simulink model "s_c_nbe_m32k"  (R2018a)
settings: Solver=VariableStepDiscrete  StartTime=0.0  StopTime=1000  RelTol=1e-3
undefined symbols (not defined in the file): fft_stages, n_taps, output_bits, pfb_coeff_gen_calc, xengbits
libraries: xbsIndex_r4 x23714, casper_library_misc x17, xps_library x4, casper_library_scopes x4, xbsReplacements_r4 x4
(part 114 of 171)

== system s_c_nbe_m32k/DDC/dec_fir_async3/fir_col_async3/fir_tap8 ==
  a : Inport
  b : Inport  Port=2
  c : Inport  Port=3
  d : Inport  Port=4
  dv_in : Inport  Port=5
  AddSub0 : xbsIndex_r4/AddSub  mode=Addition  use_carryin=off  use_carryout=off  en=on  latency=add_latency  precision=Full  arith_type="Signed  (2's comp)"  n_bits=18  bin_pt=16  quantization=Truncate  overflow=Wrap  use_behavioral_HDL=on  hw_selection=Fabric  pipelined=off  use_rpm=on  dbl_ovrd=off  block_type=addsub
  AddSub1 : xbsIndex_r4/AddSub  mode=Addition  use_carryin=off  use_carryout=off  en=on  latency=add_latency  precision=Full  arith_type="Signed  (2's comp)"  n_bits=18  bin_pt=16  quantization=Truncate  overflow=Wrap  use_behavioral_HDL=on  hw_selection=Fabric  pipelined=off  use_rpm=on  dbl_ovrd=off  block_type=addsub
  Mult0 : xbsIndex_r4/Mult  precision=Full  arith_type="Signed  (2's comp)"  n_bits=18  bin_pt=17  quantization=Truncate  overflow=Wrap  en=on  latency=mult_latency  use_behavioral_HDL=on  opt=Speed  use_embedded=on  optimum_pipeline=off  pipeline=on  dbl_ovrd=off  use_rpm=off  placement_style=Rectangular shape  block_type=mult
  Mult1 : xbsIndex_r4/Mult  precision=Full  arith_type="Signed  (2's comp)"  n_bits=18  bin_pt=17  quantization=Truncate  overflow=Wrap  en=on  latency=mult_latency  use_behavioral_HDL=on  opt=Speed  use_embedded=on  optimum_pipeline=off  pipeline=on  dbl_ovrd=off  use_rpm=off  placement_style=Rectangular shape  block_type=mult
  Register{0..3} (4 alike) : xbsIndex_r4/Register  init=0  rst=off  en=on  dbl_ovrd=off  block_type=register
  coefficient : xbsIndex_r4/Constant  const=factor  gui_display_data_type=Fixed-point  arith_type=Signed (2's comp)  n_bits=coeff_bit_width  bin_pt=coeff_bin_pt  preci_type=Single  exp_width=8  frac_width=24  explicit_period=on  period=1  equ=P=C  opselect=C  inp2=PCIN>>17  opr=+  inp1=P  carry=CIN  dbl_ovrd=off  block_type=constant
  a_out : Outport
  b_out : Outport  Port=2
  c_out : Outport  Port=3
  d_out : Outport  Port=4
  real : Outport  Port=5
  imag : Outport  Port=6
  wires:
  dv_in/1 -> Register0/2, Register1/2, Register2/2, Register3/2, AddSub0/3, AddSub1/3, Mult0/3, Mult1/3
  d/1 -> AddSub1/2, Register3/1
  c/1 -> AddSub0/2, Register2/1
  b/1 -> AddSub1/1, Register1/1
  a/1 -> AddSub0/1, Register0/1
  Register0/1 -> a_out/1
  Register1/1 -> b_out/1
  Register2/1 -> c_out/1
  coefficient/1 -> Mult0/1, Mult1/1
  Register3/1 -> d_out/1
  AddSub0/1 -> Mult0/2
  Mult0/1 -> real/1
  AddSub1/1 -> Mult1/2
  Mult1/1 -> imag/1

== system s_c_nbe_m32k/DDC/dec_fir_async3/fir_col_async3/fir_tap9 ==
  a : Inport
  b : Inport  Port=2
  c : Inport  Port=3
  d : Inport  Port=4
  dv_in : Inport  Port=5
  AddSub0 : xbsIndex_r4/AddSub  mode=Addition  use_carryin=off  use_carryout=off  en=on  latency=add_latency  precision=Full  arith_type="Signed  (2's comp)"  n_bits=18  bin_pt=16  quantization=Truncate  overflow=Wrap  use_behavioral_HDL=on  hw_selection=Fabric  pipelined=off  use_rpm=on  dbl_ovrd=off  block_type=addsub
  AddSub1 : xbsIndex_r4/AddSub  mode=Addition  use_carryin=off  use_carryout=off  en=on  latency=add_latency  precision=Full  arith_type="Signed  (2's comp)"  n_bits=18  bin_pt=16  quantization=Truncate  overflow=Wrap  use_behavioral_HDL=on  hw_selection=Fabric  pipelined=off  use_rpm=on  dbl_ovrd=off  block_type=addsub
  Mult0 : xbsIndex_r4/Mult  precision=Full  arith_type="Signed  (2's comp)"  n_bits=18  bin_pt=17  quantization=Truncate  overflow=Wrap  en=on  latency=mult_latency  use_behavioral_HDL=on  opt=Speed  use_embedded=on  optimum_pipeline=off  pipeline=on  dbl_ovrd=off  use_rpm=off  placement_style=Rectangular shape  block_type=mult
  Mult1 : xbsIndex_r4/Mult  precision=Full  arith_type="Signed  (2's comp)"  n_bits=18  bin_pt=17  quantization=Truncate  overflow=Wrap  en=on  latency=mult_latency  use_behavioral_HDL=on  opt=Speed  use_embedded=on  optimum_pipeline=off  pipeline=on  dbl_ovrd=off  use_rpm=off  placement_style=Rectangular shape  block_type=mult
  Register{0..3} (4 alike) : xbsIndex_r4/Register  init=0  rst=off  en=on  dbl_ovrd=off  block_type=register
  coefficient : xbsIndex_r4/Constant  const=factor  gui_display_data_type=Fixed-point  arith_type=Signed (2's comp)  n_bits=coeff_bit_width  bin_pt=coeff_bin_pt  preci_type=Single  exp_width=8  frac_width=24  explicit_period=on  period=1  equ=P=C  opselect=C  inp2=PCIN>>17  opr=+  inp1=P  carry=CIN  dbl_ovrd=off  block_type=constant
  a_out : Outport
  b_out : Outport  Port=2
  c_out : Outport  Port=3
  d_out : Outport  Port=4
  real : Outport  Port=5
  imag : Outport  Port=6
  wires:
  dv_in/1 -> Register0/2, Register1/2, Register2/2, Register3/2, AddSub0/3, AddSub1/3, Mult0/3, Mult1/3
  d/1 -> AddSub1/2, Register3/1
  c/1 -> AddSub0/2, Register2/1
  b/1 -> AddSub1/1, Register1/1
  a/1 -> AddSub0/1, Register0/1
  Register0/1 -> a_out/1
  Register1/1 -> b_out/1
  Register2/1 -> c_out/1
  coefficient/1 -> Mult0/1, Mult1/1
  Register3/1 -> d_out/1
  AddSub0/1 -> Mult0/2
  Mult0/1 -> real/1
  AddSub1/1 -> Mult1/2
  Mult1/1 -> imag/1

== system s_c_nbe_m32k/DDC/dec_fir_async3/fir_col_async4/adder_tree1 ==
  sync : Inport
  din1 : Inport  Port=2
  din2 : Inport  Port=3
  din3 : Inport  Port=4
  din4 : Inport  Port=5
  din5 : Inport  Port=6
  din6 : Inport  Port=7
  din7 : Inport  Port=8
  din8 : Inport  Port=9
  din9 : Inport  Port=10
  din10 : Inport  Port=11
  din11 : Inport  Port=12
  din12 : Inport  Port=13
  din13 : Inport  Port=14
  din14 : Inport  Port=15
  din15 : Inport  Port=16
  din16 : Inport  Port=17
  addr{1..8} (8 alike) : xbsIndex_r4/AddSub  mode=Addition  use_carryin=off  use_carryout=off  en=off  latency=7  precision=Full  arith_type=Unsigned  n_bits=16  bin_pt=14  quantization=Truncate  overflow=Wrap  use_behavioral_HDL=on  hw_selection=DSP48  pipelined=on  use_rpm=on  dbl_ovrd=off  block_type=addsub
  addr{9..15} (7 alike) : xbsIndex_r4/AddSub  mode=Addition  use_carryin=off  use_carryout=off  en=off  latency=7  precision=Full  arith_type=Unsigned  n_bits=16  bin_pt=14  quantization=Truncate  overflow=Wrap  use_behavioral_HDL=off  hw_selection=DSP48  pipelined=on  use_rpm=on  dbl_ovrd=off  block_type=addsub
  sync_delay : xbsIndex_r4/Delay  rst=off  infoeditControl=Selection of Reset will increase slice count due to use of real FFs and instead of SRLs  en=off  latency=28  reg_retiming=on  dbl_ovrd=off  block_type=delay
      settings: block_version=11.4
  sync_out : Outport
  dout : Outport  Port=2
  wires:
  sync/1 -> sync_delay/1
  sync_delay/1 -> sync_out/1
  din1/1 -> addr1/1
  din2/1 -> addr1/2
  din3/1 -> addr2/1
  din4/1 -> addr2/2
  din5/1 -> addr3/1
  din6/1 -> addr3/2
  din7/1 -> addr4/1
  din8/1 -> addr4/2
  din9/1 -> addr5/1
  din10/1 -> addr5/2
  din11/1 -> addr6/1
  din12/1 -> addr6/2
  din13/1 -> addr7/1
  din14/1 -> addr7/2
  din15/1 -> addr8/1
  din16/1 -> addr8/2
  addr1/1 -> addr9/1
  addr2/1 -> addr9/2
  addr3/1 -> addr10/1
  addr4/1 -> addr10/2
  addr5/1 -> addr11/1
  addr6/1 -> addr11/2
  addr7/1 -> addr12/1
  addr8/1 -> addr12/2
  addr9/1 -> addr13/1
  addr10/1 -> addr13/2
  addr11/1 -> addr14/1
  addr12/1 -> addr14/2
  addr13/1 -> addr15/1
  addr14/1 -> addr15/2
  addr15/1 -> dout/1

== system s_c_nbe_m32k/DDC/dec_fir_async3/fir_col_async4/adder_tree2 ==
  sync : Inport
  din1 : Inport  Port=2
  din2 : Inport  Port=3
  din3 : Inport  Port=4
  din4 : Inport  Port=5
  din5 : Inport  Port=6
  din6 : Inport  Port=7
  din7 : Inport  Port=8
  din8 : Inport  Port=9
  din9 : Inport  Port=10
  din10 : Inport  Port=11
  din11 : Inport  Port=12
  din12 : Inport  Port=13
  din13 : Inport  Port=14
  din14 : Inport  Port=15
  din15 : Inport  Port=16
  din16 : Inport  Port=17
  addr{1..8} (8 alike) : xbsIndex_r4/AddSub  mode=Addition  use_carryin=off  use_carryout=off  en=off  latency=7  precision=Full  arith_type=Unsigned  n_bits=16  bin_pt=14  quantization=Truncate  overflow=Wrap  use_behavioral_HDL=on  hw_selection=DSP48  pipelined=on  use_rpm=on  dbl_ovrd=off  block_type=addsub
  addr{9..15} (7 alike) : xbsIndex_r4/AddSub  mode=Addition  use_carryin=off  use_carryout=off  en=off  latency=7  precision=Full  arith_type=Unsigned  n_bits=16  bin_pt=14  quantization=Truncate  overflow=Wrap  use_behavioral_HDL=off  hw_selection=DSP48  pipelined=on  use_rpm=on  dbl_ovrd=off  block_type=addsub
  sync_delay : xbsIndex_r4/Delay  rst=off  infoeditControl=Selection of Reset will increase slice count due to use of real FFs and instead of SRLs  en=off  latency=28  reg_retiming=on  dbl_ovrd=off  block_type=delay
      settings: block_version=11.4
  sync_out : Outport
  dout : Outport  Port=2
  wires:
  sync/1 -> sync_delay/1
  sync_delay/1 -> sync_out/1
  din1/1 -> addr1/1
  din2/1 -> addr1/2
  din3/1 -> addr2/1
  din4/1 -> addr2/2
  din5/1 -> addr3/1
  din6/1 -> addr3/2
  din7/1 -> addr4/1
  din8/1 -> addr4/2
  din9/1 -> addr5/1
  din10/1 -> addr5/2
  din11/1 -> addr6/1
  din12/1 -> addr6/2
  din13/1 -> addr7/1
  din14/1 -> addr7/2
  din15/1 -> addr8/1
  din16/1 -> addr8/2
  addr1/1 -> addr9/1
  addr2/1 -> addr9/2
  addr3/1 -> addr10/1
  addr4/1 -> addr10/2
  addr5/1 -> addr11/1
  addr6/1 -> addr11/2
  addr7/1 -> addr12/1
  addr8/1 -> addr12/2
  addr9/1 -> addr13/1
  addr10/1 -> addr13/2
  addr11/1 -> addr14/1
  addr12/1 -> addr14/2
  addr13/1 -> addr15/1
  addr14/1 -> addr15/2
  addr15/1 -> dout/1

== system s_c_nbe_m32k/DDC/dec_fir_async3/fir_col_async4/fir_tap1 ==
  a : Inport
  b : Inport  Port=2
  c : Inport  Port=3
  d : Inport  Port=4
  dv_in : Inport  Port=5
  AddSub0 : xbsIndex_r4/AddSub  mode=Addition  use_carryin=off  use_carryout=off  en=on  latency=add_latency  precision=Full  arith_type="Signed  (2's comp)"  n_bits=18  bin_pt=16  quantization=Truncate  overflow=Wrap  use_behavioral_HDL=on  hw_selection=Fabric  pipelined=off  use_rpm=on  dbl_ovrd=off  block_type=addsub
  AddSub1 : xbsIndex_r4/AddSub  mode=Addition  use_carryin=off  use_carryout=off  en=on  latency=add_latency  precision=Full  arith_type="Signed  (2's comp)"  n_bits=18  bin_pt=16  quantization=Truncate  overflow=Wrap  use_behavioral_HDL=on  hw_selection=Fabric  pipelined=off  use_rpm=on  dbl_ovrd=off  block_type=addsub
  Mult0 : xbsIndex_r4/Mult  precision=Full  arith_type="Signed  (2's comp)"  n_bits=18  bin_pt=17  quantization=Truncate  overflow=Wrap  en=on  latency=mult_latency  use_behavioral_HDL=on  opt=Speed  use_embedded=on  optimum_pipeline=off  pipeline=on  dbl_ovrd=off  use_rpm=off  placement_style=Rectangular shape  block_type=mult
  Mult1 : xbsIndex_r4/Mult  precision=Full  arith_type="Signed  (2's comp)"  n_bits=18  bin_pt=17  quantization=Truncate  overflow=Wrap  en=on  latency=mult_latency  use_behavioral_HDL=on  opt=Speed  use_embedded=on  optimum_pipeline=off  pipeline=on  dbl_ovrd=off  use_rpm=off  placement_style=Rectangular shape  block_type=mult
  Register{0..3} (4 alike) : xbsIndex_r4/Register  init=0  rst=off  en=on  dbl_ovrd=off  block_type=register
  coefficient : xbsIndex_r4/Constant  const=factor  gui_display_data_type=Fixed-point  arith_type=Signed (2's comp)  n_bits=coeff_bit_width  bin_pt=coeff_bin_pt  preci_type=Single  exp_width=8  frac_width=24  explicit_period=on  period=1  equ=P=C  opselect=C  inp2=PCIN>>17  opr=+  inp1=P  carry=CIN  dbl_ovrd=off  block_type=constant
  a_out : Outport
  b_out : Outport  Port=2
  c_out : Outport  Port=3
  d_out : Outport  Port=4
  real : Outport  Port=5
  imag : Outport  Port=6
  wires:
  dv_in/1 -> Register0/2, Register1/2, Register2/2, Register3/2, AddSub0/3, AddSub1/3, Mult0/3, Mult1/3
  d/1 -> AddSub1/2, Register3/1
  c/1 -> AddSub0/2, Register2/1
  b/1 -> AddSub1/1, Register1/1
  a/1 -> AddSub0/1, Register0/1
  Register0/1 -> a_out/1
  Register1/1 -> b_out/1
  Register2/1 -> c_out/1
  coefficient/1 -> Mult0/1, Mult1/1
  Register3/1 -> d_out/1
  AddSub0/1 -> Mult0/2
  Mult0/1 -> real/1
  AddSub1/1 -> Mult1/2
  Mult1/1 -> imag/1

== system s_c_nbe_m32k/DDC/dec_fir_async3/fir_col_async4/fir_tap10 ==
  a : Inport
  b : Inport  Port=2
  c : Inport  Port=3
  d : Inport  Port=4
  dv_in : Inport  Port=5
  AddSub0 : xbsIndex_r4/AddSub  mode=Addition  use_carryin=off  use_carryout=off  en=on  latency=add_latency  precision=Full  arith_type="Signed  (2's comp)"  n_bits=18  bin_pt=16  quantization=Truncate  overflow=Wrap  use_behavioral_HDL=on  hw_selection=Fabric  pipelined=off  use_rpm=on  dbl_ovrd=off  block_type=addsub
  AddSub1 : xbsIndex_r4/AddSub  mode=Addition  use_carryin=off  use_carryout=off  en=on  latency=add_latency  precision=Full  arith_type="Signed  (2's comp)"  n_bits=18  bin_pt=16  quantization=Truncate  overflow=Wrap  use_behavioral_HDL=on  hw_selection=Fabric  pipelined=off  use_rpm=on  dbl_ovrd=off  block_type=addsub
  Mult0 : xbsIndex_r4/Mult  precision=Full  arith_type="Signed  (2's comp)"  n_bits=18  bin_pt=17  quantization=Truncate  overflow=Wrap  en=on  latency=mult_latency  use_behavioral_HDL=on  opt=Speed  use_embedded=on  optimum_pipeline=off  pipeline=on  dbl_ovrd=off  use_rpm=off  placement_style=Rectangular shape  block_type=mult
  Mult1 : xbsIndex_r4/Mult  precision=Full  arith_type="Signed  (2's comp)"  n_bits=18  bin_pt=17  quantization=Truncate  overflow=Wrap  en=on  latency=mult_latency  use_behavioral_HDL=on  opt=Speed  use_embedded=on  optimum_pipeline=off  pipeline=on  dbl_ovrd=off  use_rpm=off  placement_style=Rectangular shape  block_type=mult
  Register{0..3} (4 alike) : xbsIndex_r4/Register  init=0  rst=off  en=on  dbl_ovrd=off  block_type=register
  coefficient : xbsIndex_r4/Constant  const=factor  gui_display_data_type=Fixed-point  arith_type=Signed (2's comp)  n_bits=coeff_bit_width  bin_pt=coeff_bin_pt  preci_type=Single  exp_width=8  frac_width=24  explicit_period=on  period=1  equ=P=C  opselect=C  inp2=PCIN>>17  opr=+  inp1=P  carry=CIN  dbl_ovrd=off  block_type=constant
  a_out : Outport
  b_out : Outport  Port=2
  c_out : Outport  Port=3
  d_out : Outport  Port=4
  real : Outport  Port=5
  imag : Outport  Port=6
  wires:
  dv_in/1 -> Register0/2, Register1/2, Register2/2, Register3/2, AddSub0/3, AddSub1/3, Mult0/3, Mult1/3
  d/1 -> AddSub1/2, Register3/1
  c/1 -> AddSub0/2, Register2/1
  b/1 -> AddSub1/1, Register1/1
  a/1 -> AddSub0/1, Register0/1
  Register0/1 -> a_out/1
  Register1/1 -> b_out/1
  Register2/1 -> c_out/1
  coefficient/1 -> Mult0/1, Mult1/1
  Register3/1 -> d_out/1
  AddSub0/1 -> Mult0/2
  Mult0/1 -> real/1
  AddSub1/1 -> Mult1/2
  Mult1/1 -> imag/1

== system s_c_nbe_m32k/DDC/dec_fir_async3/fir_col_async4/fir_tap11 ==
  a : Inport
  b : Inport  Port=2
  c : Inport  Port=3
  d : Inport  Port=4
  dv_in : Inport  Port=5
  AddSub0 : xbsIndex_r4/AddSub  mode=Addition  use_carryin=off  use_carryout=off  en=on  latency=add_latency  precision=Full  arith_type="Signed  (2's comp)"  n_bits=18  bin_pt=16  quantization=Truncate  overflow=Wrap  use_behavioral_HDL=on  hw_selection=Fabric  pipelined=off  use_rpm=on  dbl_ovrd=off  block_type=addsub
  AddSub1 : xbsIndex_r4/AddSub  mode=Addition  use_carryin=off  use_carryout=off  en=on  latency=add_latency  precision=Full  arith_type="Signed  (2's comp)"  n_bits=18  bin_pt=16  quantization=Truncate  overflow=Wrap  use_behavioral_HDL=on  hw_selection=Fabric  pipelined=off  use_rpm=on  dbl_ovrd=off  block_type=addsub
  Mult0 : xbsIndex_r4/Mult  precision=Full  arith_type="Signed  (2's comp)"  n_bits=18  bin_pt=17  quantization=Truncate  overflow=Wrap  en=on  latency=mult_latency  use_behavioral_HDL=on  opt=Speed  use_embedded=on  optimum_pipeline=off  pipeline=on  dbl_ovrd=off  use_rpm=off  placement_style=Rectangular shape  block_type=mult
  Mult1 : xbsIndex_r4/Mult  precision=Full  arith_type="Signed  (2's comp)"  n_bits=18  bin_pt=17  quantization=Truncate  overflow=Wrap  en=on  latency=mult_latency  use_behavioral_HDL=on  opt=Speed  use_embedded=on  optimum_pipeline=off  pipeline=on  dbl_ovrd=off  use_rpm=off  placement_style=Rectangular shape  block_type=mult
  Register{0..3} (4 alike) : xbsIndex_r4/Register  init=0  rst=off  en=on  dbl_ovrd=off  block_type=register
  coefficient : xbsIndex_r4/Constant  const=factor  gui_display_data_type=Fixed-point  arith_type=Signed (2's comp)  n_bits=coeff_bit_width  bin_pt=coeff_bin_pt  preci_type=Single  exp_width=8  frac_width=24  explicit_period=on  period=1  equ=P=C  opselect=C  inp2=PCIN>>17  opr=+  inp1=P  carry=CIN  dbl_ovrd=off  block_type=constant
  a_out : Outport
  b_out : Outport  Port=2
  c_out : Outport  Port=3
  d_out : Outport  Port=4
  real : Outport  Port=5
  imag : Outport  Port=6
  wires:
  dv_in/1 -> Register0/2, Register1/2, Register2/2, Register3/2, AddSub0/3, AddSub1/3, Mult0/3, Mult1/3
  d/1 -> AddSub1/2, Register3/1
  c/1 -> AddSub0/2, Register2/1
  b/1 -> AddSub1/1, Register1/1
  a/1 -> AddSub0/1, Register0/1
  Register0/1 -> a_out/1
  Register1/1 -> b_out/1
  Register2/1 -> c_out/1
  coefficient/1 -> Mult0/1, Mult1/1
  Register3/1 -> d_out/1
  AddSub0/1 -> Mult0/2
  Mult0/1 -> real/1
  AddSub1/1 -> Mult1/2
  Mult1/1 -> imag/1

== system s_c_nbe_m32k/DDC/dec_fir_async3/fir_col_async4/fir_tap12 ==
  a : Inport
  b : Inport  Port=2
  c : Inport  Port=3
  d : Inport  Port=4
  dv_in : Inport  Port=5
  AddSub0 : xbsIndex_r4/AddSub  mode=Addition  use_carryin=off  use_carryout=off  en=on  latency=add_latency  precision=Full  arith_type="Signed  (2's comp)"  n_bits=18  bin_pt=16  quantization=Truncate  overflow=Wrap  use_behavioral_HDL=on  hw_selection=Fabric  pipelined=off  use_rpm=on  dbl_ovrd=off  block_type=addsub
  AddSub1 : xbsIndex_r4/AddSub  mode=Addition  use_carryin=off  use_carryout=off  en=on  latency=add_latency  precision=Full  arith_type="Signed  (2's comp)"  n_bits=18  bin_pt=16  quantization=Truncate  overflow=Wrap  use_behavioral_HDL=on  hw_selection=Fabric  pipelined=off  use_rpm=on  dbl_ovrd=off  block_type=addsub
  Mult0 : xbsIndex_r4/Mult  precision=Full  arith_type="Signed  (2's comp)"  n_bits=18  bin_pt=17  quantization=Truncate  overflow=Wrap  en=on  latency=mult_latency  use_behavioral_HDL=on  opt=Speed  use_embedded=on  optimum_pipeline=off  pipeline=on  dbl_ovrd=off  use_rpm=off  placement_style=Rectangular shape  block_type=mult
  Mult1 : xbsIndex_r4/Mult  precision=Full  arith_type="Signed  (2's comp)"  n_bits=18  bin_pt=17  quantization=Truncate  overflow=Wrap  en=on  latency=mult_latency  use_behavioral_HDL=on  opt=Speed  use_embedded=on  optimum_pipeline=off  pipeline=on  dbl_ovrd=off  use_rpm=off  placement_style=Rectangular shape  block_type=mult
  Register{0..3} (4 alike) : xbsIndex_r4/Register  init=0  rst=off  en=on  dbl_ovrd=off  block_type=register
  coefficient : xbsIndex_r4/Constant  const=factor  gui_display_data_type=Fixed-point  arith_type=Signed (2's comp)  n_bits=coeff_bit_width  bin_pt=coeff_bin_pt  preci_type=Single  exp_width=8  frac_width=24  explicit_period=on  period=1  equ=P=C  opselect=C  inp2=PCIN>>17  opr=+  inp1=P  carry=CIN  dbl_ovrd=off  block_type=constant
  a_out : Outport
  b_out : Outport  Port=2
  c_out : Outport  Port=3
  d_out : Outport  Port=4
  real : Outport  Port=5
  imag : Outport  Port=6
  wires:
  dv_in/1 -> Register0/2, Register1/2, Register2/2, Register3/2, AddSub0/3, AddSub1/3, Mult0/3, Mult1/3
  d/1 -> AddSub1/2, Register3/1
  c/1 -> AddSub0/2, Register2/1
  b/1 -> AddSub1/1, Register1/1
  a/1 -> AddSub0/1, Register0/1
  Register0/1 -> a_out/1
  Register1/1 -> b_out/1
  Register2/1 -> c_out/1
  coefficient/1 -> Mult0/1, Mult1/1
  Register3/1 -> d_out/1
  AddSub0/1 -> Mult0/2
  Mult0/1 -> real/1
  AddSub1/1 -> Mult1/2
  Mult1/1 -> imag/1

== system s_c_nbe_m32k/DDC/dec_fir_async3/fir_col_async4/fir_tap13 ==
  a : Inport
  b : Inport  Port=2
  c : Inport  Port=3
  d : Inport  Port=4
  dv_in : Inport  Port=5
  AddSub0 : xbsIndex_r4/AddSub  mode=Addition  use_carryin=off  use_carryout=off  en=on  latency=add_latency  precision=Full  arith_type="Signed  (2's comp)"  n_bits=18  bin_pt=16  quantization=Truncate  overflow=Wrap  use_behavioral_HDL=on  hw_selection=Fabric  pipelined=off  use_rpm=on  dbl_ovrd=off  block_type=addsub
  AddSub1 : xbsIndex_r4/AddSub  mode=Addition  use_carryin=off  use_carryout=off  en=on  latency=add_latency  precision=Full  arith_type="Signed  (2's comp)"  n_bits=18  bin_pt=16  quantization=Truncate  overflow=Wrap  use_behavioral_HDL=on  hw_selection=Fabric  pipelined=off  use_rpm=on  dbl_ovrd=off  block_type=addsub
  Mult0 : xbsIndex_r4/Mult  precision=Full  arith_type="Signed  (2's comp)"  n_bits=18  bin_pt=17  quantization=Truncate  overflow=Wrap  en=on  latency=mult_latency  use_behavioral_HDL=on  opt=Speed  use_embedded=on  optimum_pipeline=off  pipeline=on  dbl_ovrd=off  use_rpm=off  placement_style=Rectangular shape  block_type=mult
  Mult1 : xbsIndex_r4/Mult  precision=Full  arith_type="Signed  (2's comp)"  n_bits=18  bin_pt=17  quantization=Truncate  overflow=Wrap  en=on  latency=mult_latency  use_behavioral_HDL=on  opt=Speed  use_embedded=on  optimum_pipeline=off  pipeline=on  dbl_ovrd=off  use_rpm=off  placement_style=Rectangular shape  block_type=mult
  Register{0..3} (4 alike) : xbsIndex_r4/Register  init=0  rst=off  en=on  dbl_ovrd=off  block_type=register
  coefficient : xbsIndex_r4/Constant  const=factor  gui_display_data_type=Fixed-point  arith_type=Signed (2's comp)  n_bits=coeff_bit_width  bin_pt=coeff_bin_pt  preci_type=Single  exp_width=8  frac_width=24  explicit_period=on  period=1  equ=P=C  opselect=C  inp2=PCIN>>17  opr=+  inp1=P  carry=CIN  dbl_ovrd=off  block_type=constant
  a_out : Outport
  b_out : Outport  Port=2
  c_out : Outport  Port=3
  d_out : Outport  Port=4
  real : Outport  Port=5
  imag : Outport  Port=6
  wires:
  dv_in/1 -> Register0/2, Register1/2, Register2/2, Register3/2, AddSub0/3, AddSub1/3, Mult0/3, Mult1/3
  d/1 -> AddSub1/2, Register3/1
  c/1 -> AddSub0/2, Register2/1
  b/1 -> AddSub1/1, Register1/1
  a/1 -> AddSub0/1, Register0/1
  Register0/1 -> a_out/1
  Register1/1 -> b_out/1
  Register2/1 -> c_out/1
  coefficient/1 -> Mult0/1, Mult1/1
  Register3/1 -> d_out/1
  AddSub0/1 -> Mult0/2
  Mult0/1 -> real/1
  AddSub1/1 -> Mult1/2
  Mult1/1 -> imag/1

== system s_c_nbe_m32k/DDC/dec_fir_async3/fir_col_async4/fir_tap14 ==
  a : Inport
  b : Inport  Port=2
  c : Inport  Port=3
  d : Inport  Port=4
  dv_in : Inport  Port=5
  AddSub0 : xbsIndex_r4/AddSub  mode=Addition  use_carryin=off  use_carryout=off  en=on  latency=add_latency  precision=Full  arith_type="Signed  (2's comp)"  n_bits=18  bin_pt=16  quantization=Truncate  overflow=Wrap  use_behavioral_HDL=on  hw_selection=Fabric  pipelined=off  use_rpm=on  dbl_ovrd=off  block_type=addsub
  AddSub1 : xbsIndex_r4/AddSub  mode=Addition  use_carryin=off  use_carryout=off  en=on  latency=add_latency  precision=Full  arith_type="Signed  (2's comp)"  n_bits=18  bin_pt=16  quantization=Truncate  overflow=Wrap  use_behavioral_HDL=on  hw_selection=Fabric  pipelined=off  use_rpm=on  dbl_ovrd=off  block_type=addsub
  Mult0 : xbsIndex_r4/Mult  precision=Full  arith_type="Signed  (2's comp)"  n_bits=18  bin_pt=17  quantization=Truncate  overflow=Wrap  en=on  latency=mult_latency  use_behavioral_HDL=on  opt=Speed  use_embedded=on  optimum_pipeline=off  pipeline=on  dbl_ovrd=off  use_rpm=off  placement_style=Rectangular shape  block_type=mult
  Mult1 : xbsIndex_r4/Mult  precision=Full  arith_type="Signed  (2's comp)"  n_bits=18  bin_pt=17  quantization=Truncate  overflow=Wrap  en=on  latency=mult_latency  use_behavioral_HDL=on  opt=Speed  use_embedded=on  optimum_pipeline=off  pipeline=on  dbl_ovrd=off  use_rpm=off  placement_style=Rectangular shape  block_type=mult
  Register{0..3} (4 alike) : xbsIndex_r4/Register  init=0  rst=off  en=on  dbl_ovrd=off  block_type=register
  coefficient : xbsIndex_r4/Constant  const=factor  gui_display_data_type=Fixed-point  arith_type=Signed (2's comp)  n_bits=coeff_bit_width  bin_pt=coeff_bin_pt  preci_type=Single  exp_width=8  frac_width=24  explicit_period=on  period=1  equ=P=C  opselect=C  inp2=PCIN>>17  opr=+  inp1=P  carry=CIN  dbl_ovrd=off  block_type=constant
  a_out : Outport
  b_out : Outport  Port=2
  c_out : Outport  Port=3
  d_out : Outport  Port=4
  real : Outport  Port=5
  imag : Outport  Port=6
  wires:
  dv_in/1 -> Register0/2, Register1/2, Register2/2, Register3/2, AddSub0/3, AddSub1/3, Mult0/3, Mult1/3
  d/1 -> AddSub1/2, Register3/1
  c/1 -> AddSub0/2, Register2/1
  b/1 -> AddSub1/1, Register1/1
  a/1 -> AddSub0/1, Register0/1
  Register0/1 -> a_out/1
  Register1/1 -> b_out/1
  Register2/1 -> c_out/1
  coefficient/1 -> Mult0/1, Mult1/1
  Register3/1 -> d_out/1
  AddSub0/1 -> Mult0/2
  Mult0/1 -> real/1
  AddSub1/1 -> Mult1/2
  Mult1/1 -> imag/1

== system s_c_nbe_m32k/DDC/dec_fir_async3/fir_col_async4/fir_tap15 ==
  a : Inport
  b : Inport  Port=2
  c : Inport  Port=3
  d : Inport  Port=4
  dv_in : Inport  Port=5
  AddSub0 : xbsIndex_r4/AddSub  mode=Addition  use_carryin=off  use_carryout=off  en=on  latency=add_latency  precision=Full  arith_type="Signed  (2's comp)"  n_bits=18  bin_pt=16  quantization=Truncate  overflow=Wrap  use_behavioral_HDL=on  hw_selection=Fabric  pipelined=off  use_rpm=on  dbl_ovrd=off  block_type=addsub
  AddSub1 : xbsIndex_r4/AddSub  mode=Addition  use_carryin=off  use_carryout=off  en=on  latency=add_latency  precision=Full  arith_type="Signed  (2's comp)"  n_bits=18  bin_pt=16  quantization=Truncate  overflow=Wrap  use_behavioral_HDL=on  hw_selection=Fabric  pipelined=off  use_rpm=on  dbl_ovrd=off  block_type=addsub
  Mult0 : xbsIndex_r4/Mult  precision=Full  arith_type="Signed  (2's comp)"  n_bits=18  bin_pt=17  quantization=Truncate  overflow=Wrap  en=on  latency=mult_latency  use_behavioral_HDL=on  opt=Speed  use_embedded=on  optimum_pipeline=off  pipeline=on  dbl_ovrd=off  use_rpm=off  placement_style=Rectangular shape  block_type=mult
  Mult1 : xbsIndex_r4/Mult  precision=Full  arith_type="Signed  (2's comp)"  n_bits=18  bin_pt=17  quantization=Truncate  overflow=Wrap  en=on  latency=mult_latency  use_behavioral_HDL=on  opt=Speed  use_embedded=on  optimum_pipeline=off  pipeline=on  dbl_ovrd=off  use_rpm=off  placement_style=Rectangular shape  block_type=mult
  Register{0..3} (4 alike) : xbsIndex_r4/Register  init=0  rst=off  en=on  dbl_ovrd=off  block_type=register
  coefficient : xbsIndex_r4/Constant  const=factor  gui_display_data_type=Fixed-point  arith_type=Signed (2's comp)  n_bits=coeff_bit_width  bin_pt=coeff_bin_pt  preci_type=Single  exp_width=8  frac_width=24  explicit_period=on  period=1  equ=P=C  opselect=C  inp2=PCIN>>17  opr=+  inp1=P  carry=CIN  dbl_ovrd=off  block_type=constant
  a_out : Outport
  b_out : Outport  Port=2
  c_out : Outport  Port=3
  d_out : Outport  Port=4
  real : Outport  Port=5
  imag : Outport  Port=6
  wires:
  dv_in/1 -> Register0/2, Register1/2, Register2/2, Register3/2, AddSub0/3, AddSub1/3, Mult0/3, Mult1/3
  d/1 -> AddSub1/2, Register3/1
  c/1 -> AddSub0/2, Register2/1
  b/1 -> AddSub1/1, Register1/1
  a/1 -> AddSub0/1, Register0/1
  Register0/1 -> a_out/1
  Register1/1 -> b_out/1
  Register2/1 -> c_out/1
  coefficient/1 -> Mult0/1, Mult1/1
  Register3/1 -> d_out/1
  AddSub0/1 -> Mult0/2
  Mult0/1 -> real/1
  AddSub1/1 -> Mult1/2
  Mult1/1 -> imag/1

== system s_c_nbe_m32k/DDC/dec_fir_async3/fir_col_async4/fir_tap16 ==
  a : Inport
  b : Inport  Port=2
  c : Inport  Port=3
  d : Inport  Port=4
  dv_in : Inport  Port=5
  AddSub0 : xbsIndex_r4/AddSub  mode=Addition  use_carryin=off  use_carryout=off  en=on  latency=add_latency  precision=Full  arith_type="Signed  (2's comp)"  n_bits=18  bin_pt=16  quantization=Truncate  overflow=Wrap  use_behavioral_HDL=on  hw_selection=Fabric  pipelined=off  use_rpm=on  dbl_ovrd=off  block_type=addsub
  AddSub1 : xbsIndex_r4/AddSub  mode=Addition  use_carryin=off  use_carryout=off  en=on  latency=add_latency  precision=Full  arith_type="Signed  (2's comp)"  n_bits=18  bin_pt=16  quantization=Truncate  overflow=Wrap  use_behavioral_HDL=on  hw_selection=Fabric  pipelined=off  use_rpm=on  dbl_ovrd=off  block_type=addsub
  Mult0 : xbsIndex_r4/Mult  precision=Full  arith_type="Signed  (2's comp)"  n_bits=18  bin_pt=17  quantization=Truncate  overflow=Wrap  en=on  latency=mult_latency  use_behavioral_HDL=on  opt=Speed  use_embedded=on  optimum_pipeline=off  pipeline=on  dbl_ovrd=off  use_rpm=off  placement_style=Rectangular shape  block_type=mult
  Mult1 : xbsIndex_r4/Mult  precision=Full  arith_type="Signed  (2's comp)"  n_bits=18  bin_pt=17  quantization=Truncate  overflow=Wrap  en=on  latency=mult_latency  use_behavioral_HDL=on  opt=Speed  use_embedded=on  optimum_pipeline=off  pipeline=on  dbl_ovrd=off  use_rpm=off  placement_style=Rectangular shape  block_type=mult
  Register{0..3} (4 alike) : xbsIndex_r4/Register  init=0  rst=off  en=on  dbl_ovrd=off  block_type=register
  coefficient : xbsIndex_r4/Constant  const=factor  gui_display_data_type=Fixed-point  arith_type=Signed (2's comp)  n_bits=coeff_bit_width  bin_pt=coeff_bin_pt  preci_type=Single  exp_width=8  frac_width=24  explicit_period=on  period=1  equ=P=C  opselect=C  inp2=PCIN>>17  opr=+  inp1=P  carry=CIN  dbl_ovrd=off  block_type=constant
  a_out : Outport
  b_out : Outport  Port=2
  c_out : Outport  Port=3
  d_out : Outport  Port=4
  real : Outport  Port=5
  imag : Outport  Port=6
  wires:
  dv_in/1 -> Register0/2, Register1/2, Register2/2, Register3/2, AddSub0/3, AddSub1/3, Mult0/3, Mult1/3
  d/1 -> AddSub1/2, Register3/1
  c/1 -> AddSub0/2, Register2/1
  b/1 -> AddSub1/1, Register1/1
  a/1 -> AddSub0/1, Register0/1
  Register0/1 -> a_out/1
  Register1/1 -> b_out/1
  Register2/1 -> c_out/1
  coefficient/1 -> Mult0/1, Mult1/1
  Register3/1 -> d_out/1
  AddSub0/1 -> Mult0/2
  Mult0/1 -> real/1
  AddSub1/1 -> Mult1/2
  Mult1/1 -> imag/1

== system s_c_nbe_m32k/DDC/dec_fir_async3/fir_col_async4/fir_tap2 ==
  a : Inport
  b : Inport  Port=2
  c : Inport  Port=3
  d : Inport  Port=4
  dv_in : Inport  Port=5
  AddSub0 : xbsIndex_r4/AddSub  mode=Addition  use_carryin=off  use_carryout=off  en=on  latency=add_latency  precision=Full  arith_type="Signed  (2's comp)"  n_bits=18  bin_pt=16  quantization=Truncate  overflow=Wrap  use_behavioral_HDL=on  hw_selection=Fabric  pipelined=off  use_rpm=on  dbl_ovrd=off  block_type=addsub
  AddSub1 : xbsIndex_r4/AddSub  mode=Addition  use_carryin=off  use_carryout=off  en=on  latency=add_latency  precision=Full  arith_type="Signed  (2's comp)"  n_bits=18  bin_pt=16  quantization=Truncate  overflow=Wrap  use_behavioral_HDL=on  hw_selection=Fabric  pipelined=off  use_rpm=on  dbl_ovrd=off  block_type=addsub
  Mult0 : xbsIndex_r4/Mult  precision=Full  arith_type="Signed  (2's comp)"  n_bits=18  bin_pt=17  quantization=Truncate  overflow=Wrap  en=on  latency=mult_latency  use_behavioral_HDL=on  opt=Speed  use_embedded=on  optimum_pipeline=off  pipeline=on  dbl_ovrd=off  use_rpm=off  placement_style=Rectangular shape  block_type=mult
  Mult1 : xbsIndex_r4/Mult  precision=Full  arith_type="Signed  (2's comp)"  n_bits=18  bin_pt=17  quantization=Truncate  overflow=Wrap  en=on  latency=mult_latency  use_behavioral_HDL=on  opt=Speed  use_embedded=on  optimum_pipeline=off  pipeline=on  dbl_ovrd=off  use_rpm=off  placement_style=Rectangular shape  block_type=mult
  Register{0..3} (4 alike) : xbsIndex_r4/Register  init=0  rst=off  en=on  dbl_ovrd=off  block_type=register
  coefficient : xbsIndex_r4/Constant  const=factor  gui_display_data_type=Fixed-point  arith_type=Signed (2's comp)  n_bits=coeff_bit_width  bin_pt=coeff_bin_pt  preci_type=Single  exp_width=8  frac_width=24  explicit_period=on  period=1  equ=P=C  opselect=C  inp2=PCIN>>17  opr=+  inp1=P  carry=CIN  dbl_ovrd=off  block_type=constant
  a_out : Outport
  b_out : Outport  Port=2
  c_out : Outport  Port=3
  d_out : Outport  Port=4
  real : Outport  Port=5
  imag : Outport  Port=6
  wires:
  dv_in/1 -> Register0/2, Register1/2, Register2/2, Register3/2, AddSub0/3, AddSub1/3, Mult0/3, Mult1/3
  d/1 -> AddSub1/2, Register3/1
  c/1 -> AddSub0/2, Register2/1
  b/1 -> AddSub1/1, Register1/1
  a/1 -> AddSub0/1, Register0/1
  Register0/1 -> a_out/1
  Register1/1 -> b_out/1
  Register2/1 -> c_out/1
  coefficient/1 -> Mult0/1, Mult1/1
  Register3/1 -> d_out/1
  AddSub0/1 -> Mult0/2
  Mult0/1 -> real/1
  AddSub1/1 -> Mult1/2
  Mult1/1 -> imag/1

== system s_c_nbe_m32k/DDC/dec_fir_async3/fir_col_async4/fir_tap3 ==
  a : Inport
  b : Inport  Port=2
  c : Inport  Port=3
  d : Inport  Port=4
  dv_in : Inport  Port=5
  AddSub0 : xbsIndex_r4/AddSub  mode=Addition  use_carryin=off  use_carryout=off  en=on  latency=add_latency  precision=Full  arith_type="Signed  (2's comp)"  n_bits=18  bin_pt=16  quantization=Truncate  overflow=Wrap  use_behavioral_HDL=on  hw_selection=Fabric  pipelined=off  use_rpm=on  dbl_ovrd=off  block_type=addsub
  AddSub1 : xbsIndex_r4/AddSub  mode=Addition  use_carryin=off  use_carryout=off  en=on  latency=add_latency  precision=Full  arith_type="Signed  (2's comp)"  n_bits=18  bin_pt=16  quantization=Truncate  overflow=Wrap  use_behavioral_HDL=on  hw_selection=Fabric  pipelined=off  use_rpm=on  dbl_ovrd=off  block_type=addsub
  Mult0 : xbsIndex_r4/Mult  precision=Full  arith_type="Signed  (2's comp)"  n_bits=18  bin_pt=17  quantization=Truncate  overflow=Wrap  en=on  latency=mult_latency  use_behavioral_HDL=on  opt=Speed  use_embedded=on  optimum_pipeline=off  pipeline=on  dbl_ovrd=off  use_rpm=off  placement_style=Rectangular shape  block_type=mult
  Mult1 : xbsIndex_r4/Mult  precision=Full  arith_type="Signed  (2's comp)"  n_bits=18  bin_pt=17  quantization=Truncate  overflow=Wrap  en=on  latency=mult_latency  use_behavioral_HDL=on  opt=Speed  use_embedded=on  optimum_pipeline=off  pipeline=on  dbl_ovrd=off  use_rpm=off  placement_style=Rectangular shape  block_type=mult
  Register{0..3} (4 alike) : xbsIndex_r4/Register  init=0  rst=off  en=on  dbl_ovrd=off  block_type=register
  coefficient : xbsIndex_r4/Constant  const=factor  gui_display_data_type=Fixed-point  arith_type=Signed (2's comp)  n_bits=coeff_bit_width  bin_pt=coeff_bin_pt  preci_type=Single  exp_width=8  frac_width=24  explicit_period=on  period=1  equ=P=C  opselect=C  inp2=PCIN>>17  opr=+  inp1=P  carry=CIN  dbl_ovrd=off  block_type=constant
  a_out : Outport
  b_out : Outport  Port=2
  c_out : Outport  Port=3
  d_out : Outport  Port=4
  real : Outport  Port=5
  imag : Outport  Port=6
  wires:
  dv_in/1 -> Register0/2, Register1/2, Register2/2, Register3/2, AddSub0/3, AddSub1/3, Mult0/3, Mult1/3
  d/1 -> AddSub1/2, Register3/1
  c/1 -> AddSub0/2, Register2/1
  b/1 -> AddSub1/1, Register1/1
  a/1 -> AddSub0/1, Register0/1
  Register0/1 -> a_out/1
  Register1/1 -> b_out/1
  Register2/1 -> c_out/1
  coefficient/1 -> Mult0/1, Mult1/1
  Register3/1 -> d_out/1
  AddSub0/1 -> Mult0/2
  Mult0/1 -> real/1
  AddSub1/1 -> Mult1/2
  Mult1/1 -> imag/1

== system s_c_nbe_m32k/DDC/dec_fir_async3/fir_col_async4/fir_tap4 ==
  a : Inport
  b : Inport  Port=2
  c : Inport  Port=3
  d : Inport  Port=4
  dv_in : Inport  Port=5
  AddSub0 : xbsIndex_r4/AddSub  mode=Addition  use_carryin=off  use_carryout=off  en=on  latency=add_latency  precision=Full  arith_type="Signed  (2's comp)"  n_bits=18  bin_pt=16  quantization=Truncate  overflow=Wrap  use_behavioral_HDL=on  hw_selection=Fabric  pipelined=off  use_rpm=on  dbl_ovrd=off  block_type=addsub
  AddSub1 : xbsIndex_r4/AddSub  mode=Addition  use_carryin=off  use_carryout=off  en=on  latency=add_latency  precision=Full  arith_type="Signed  (2's comp)"  n_bits=18  bin_pt=16  quantization=Truncate  overflow=Wrap  use_behavioral_HDL=on  hw_selection=Fabric  pipelined=off  use_rpm=on  dbl_ovrd=off  block_type=addsub
  Mult0 : xbsIndex_r4/Mult  precision=Full  arith_type="Signed  (2's comp)"  n_bits=18  bin_pt=17  quantization=Truncate  overflow=Wrap  en=on  latency=mult_latency  use_behavioral_HDL=on  opt=Speed  use_embedded=on  optimum_pipeline=off  pipeline=on  dbl_ovrd=off  use_rpm=off  placement_style=Rectangular shape  block_type=mult
  Mult1 : xbsIndex_r4/Mult  precision=Full  arith_type="Signed  (2's comp)"  n_bits=18  bin_pt=17  quantization=Truncate  overflow=Wrap  en=on  latency=mult_latency  use_behavioral_HDL=on  opt=Speed  use_embedded=on  optimum_pipeline=off  pipeline=on  dbl_ovrd=off  use_rpm=off  placement_style=Rectangular shape  block_type=mult
  Register{0..3} (4 alike) : xbsIndex_r4/Register  init=0  rst=off  en=on  dbl_ovrd=off  block_type=register
  coefficient : xbsIndex_r4/Constant  const=factor  gui_display_data_type=Fixed-point  arith_type=Signed (2's comp)  n_bits=coeff_bit_width  bin_pt=coeff_bin_pt  preci_type=Single  exp_width=8  frac_width=24  explicit_period=on  period=1  equ=P=C  opselect=C  inp2=PCIN>>17  opr=+  inp1=P  carry=CIN  dbl_ovrd=off  block_type=constant
  a_out : Outport
  b_out : Outport  Port=2
  c_out : Outport  Port=3
  d_out : Outport  Port=4
  real : Outport  Port=5
  imag : Outport  Port=6
  wires:
  dv_in/1 -> Register0/2, Register1/2, Register2/2, Register3/2, AddSub0/3, AddSub1/3, Mult0/3, Mult1/3
  d/1 -> AddSub1/2, Register3/1
  c/1 -> AddSub0/2, Register2/1
  b/1 -> AddSub1/1, Register1/1
  a/1 -> AddSub0/1, Register0/1
  Register0/1 -> a_out/1
  Register1/1 -> b_out/1
  Register2/1 -> c_out/1
  coefficient/1 -> Mult0/1, Mult1/1
  Register3/1 -> d_out/1
  AddSub0/1 -> Mult0/2
  Mult0/1 -> real/1
  AddSub1/1 -> Mult1/2
  Mult1/1 -> imag/1

== system s_c_nbe_m32k/DDC/dec_fir_async3/fir_col_async4/fir_tap5 ==
  a : Inport
  b : Inport  Port=2
  c : Inport  Port=3
  d : Inport  Port=4
  dv_in : Inport  Port=5
  AddSub0 : xbsIndex_r4/AddSub  mode=Addition  use_carryin=off  use_carryout=off  en=on  latency=add_latency  precision=Full  arith_type="Signed  (2's comp)"  n_bits=18  bin_pt=16  quantization=Truncate  overflow=Wrap  use_behavioral_HDL=on  hw_selection=Fabric  pipelined=off  use_rpm=on  dbl_ovrd=off  block_type=addsub
  AddSub1 : xbsIndex_r4/AddSub  mode=Addition  use_carryin=off  use_carryout=off  en=on  latency=add_latency  precision=Full  arith_type="Signed  (2's comp)"  n_bits=18  bin_pt=16  quantization=Truncate  overflow=Wrap  use_behavioral_HDL=on  hw_selection=Fabric  pipelined=off  use_rpm=on  dbl_ovrd=off  block_type=addsub
  Mult0 : xbsIndex_r4/Mult  precision=Full  arith_type="Signed  (2's comp)"  n_bits=18  bin_pt=17  quantization=Truncate  overflow=Wrap  en=on  latency=mult_latency  use_behavioral_HDL=on  opt=Speed  use_embedded=on  optimum_pipeline=off  pipeline=on  dbl_ovrd=off  use_rpm=off  placement_style=Rectangular shape  block_type=mult
  Mult1 : xbsIndex_r4/Mult  precision=Full  arith_type="Signed  (2's comp)"  n_bits=18  bin_pt=17  quantization=Truncate  overflow=Wrap  en=on  latency=mult_latency  use_behavioral_HDL=on  opt=Speed  use_embedded=on  optimum_pipeline=off  pipeline=on  dbl_ovrd=off  use_rpm=off  placement_style=Rectangular shape  block_type=mult
  Register{0..3} (4 alike) : xbsIndex_r4/Register  init=0  rst=off  en=on  dbl_ovrd=off  block_type=register
  coefficient : xbsIndex_r4/Constant  const=factor  gui_display_data_type=Fixed-point  arith_type=Signed (2's comp)  n_bits=coeff_bit_width  bin_pt=coeff_bin_pt  preci_type=Single  exp_width=8  frac_width=24  explicit_period=on  period=1  equ=P=C  opselect=C  inp2=PCIN>>17  opr=+  inp1=P  carry=CIN  dbl_ovrd=off  block_type=constant
  a_out : Outport
  b_out : Outport  Port=2
  c_out : Outport  Port=3
  d_out : Outport  Port=4
  real : Outport  Port=5
  imag : Outport  Port=6
  wires:
  dv_in/1 -> Register0/2, Register1/2, Register2/2, Register3/2, AddSub0/3, AddSub1/3, Mult0/3, Mult1/3
  d/1 -> AddSub1/2, Register3/1
  c/1 -> AddSub0/2, Register2/1
  b/1 -> AddSub1/1, Register1/1
  a/1 -> AddSub0/1, Register0/1
  Register0/1 -> a_out/1
  Register1/1 -> b_out/1
  Register2/1 -> c_out/1
  coefficient/1 -> Mult0/1, Mult1/1
  Register3/1 -> d_out/1
  AddSub0/1 -> Mult0/2
  Mult0/1 -> real/1
  AddSub1/1 -> Mult1/2
  Mult1/1 -> imag/1

== system s_c_nbe_m32k/DDC/dec_fir_async3/fir_col_async4/fir_tap6 ==
  a : Inport
  b : Inport  Port=2
  c : Inport  Port=3
  d : Inport  Port=4
  dv_in : Inport  Port=5
  AddSub0 : xbsIndex_r4/AddSub  mode=Addition  use_carryin=off  use_carryout=off  en=on  latency=add_latency  precision=Full  arith_type="Signed  (2's comp)"  n_bits=18  bin_pt=16  quantization=Truncate  overflow=Wrap  use_behavioral_HDL=on  hw_selection=Fabric  pipelined=off  use_rpm=on  dbl_ovrd=off  block_type=addsub
  AddSub1 : xbsIndex_r4/AddSub  mode=Addition  use_carryin=off  use_carryout=off  en=on  latency=add_latency  precision=Full  arith_type="Signed  (2's comp)"  n_bits=18  bin_pt=16  quantization=Truncate  overflow=Wrap  use_behavioral_HDL=on  hw_selection=Fabric  pipelined=off  use_rpm=on  dbl_ovrd=off  block_type=addsub
  Mult0 : xbsIndex_r4/Mult  precision=Full  arith_type="Signed  (2's comp)"  n_bits=18  bin_pt=17  quantization=Truncate  overflow=Wrap  en=on  latency=mult_latency  use_behavioral_HDL=on  opt=Speed  use_embedded=on  optimum_pipeline=off  pipeline=on  dbl_ovrd=off  use_rpm=off  placement_style=Rectangular shape  block_type=mult
  Mult1 : xbsIndex_r4/Mult  precision=Full  arith_type="Signed  (2's comp)"  n_bits=18  bin_pt=17  quantization=Truncate  overflow=Wrap  en=on  latency=mult_latency  use_behavioral_HDL=on  opt=Speed  use_embedded=on  optimum_pipeline=off  pipeline=on  dbl_ovrd=off  use_rpm=off  placement_style=Rectangular shape  block_type=mult
  Register{0..3} (4 alike) : xbsIndex_r4/Register  init=0  rst=off  en=on  dbl_ovrd=off  block_type=register
  coefficient : xbsIndex_r4/Constant  const=factor  gui_display_data_type=Fixed-point  arith_type=Signed (2's comp)  n_bits=coeff_bit_width  bin_pt=coeff_bin_pt  preci_type=Single  exp_width=8  frac_width=24  explicit_period=on  period=1  equ=P=C  opselect=C  inp2=PCIN>>17  opr=+  inp1=P  carry=CIN  dbl_ovrd=off  block_type=constant
  a_out : Outport
  b_out : Outport  Port=2
  c_out : Outport  Port=3
  d_out : Outport  Port=4
  real : Outport  Port=5
  imag : Outport  Port=6
  wires:
  dv_in/1 -> Register0/2, Register1/2, Register2/2, Register3/2, AddSub0/3, AddSub1/3, Mult0/3, Mult1/3
  d/1 -> AddSub1/2, Register3/1
  c/1 -> AddSub0/2, Register2/1
  b/1 -> AddSub1/1, Register1/1
  a/1 -> AddSub0/1, Register0/1
  Register0/1 -> a_out/1
  Register1/1 -> b_out/1
  Register2/1 -> c_out/1
  coefficient/1 -> Mult0/1, Mult1/1
  Register3/1 -> d_out/1
  AddSub0/1 -> Mult0/2
  Mult0/1 -> real/1
  AddSub1/1 -> Mult1/2
  Mult1/1 -> imag/1

== system s_c_nbe_m32k/DDC/dec_fir_async3/fir_col_async4/fir_tap7 ==
  a : Inport
  b : Inport  Port=2
  c : Inport  Port=3
  d : Inport  Port=4
  dv_in : Inport  Port=5
  AddSub0 : xbsIndex_r4/AddSub  mode=Addition  use_carryin=off  use_carryout=off  en=on  latency=add_latency  precision=Full  arith_type="Signed  (2's comp)"  n_bits=18  bin_pt=16  quantization=Truncate  overflow=Wrap  use_behavioral_HDL=on  hw_selection=Fabric  pipelined=off  use_rpm=on  dbl_ovrd=off  block_type=addsub
  AddSub1 : xbsIndex_r4/AddSub  mode=Addition  use_carryin=off  use_carryout=off  en=on  latency=add_latency  precision=Full  arith_type="Signed  (2's comp)"  n_bits=18  bin_pt=16  quantization=Truncate  overflow=Wrap  use_behavioral_HDL=on  hw_selection=Fabric  pipelined=off  use_rpm=on  dbl_ovrd=off  block_type=addsub
  Mult0 : xbsIndex_r4/Mult  precision=Full  arith_type="Signed  (2's comp)"  n_bits=18  bin_pt=17  quantization=Truncate  overflow=Wrap  en=on  latency=mult_latency  use_behavioral_HDL=on  opt=Speed  use_embedded=on  optimum_pipeline=off  pipeline=on  dbl_ovrd=off  use_rpm=off  placement_style=Rectangular shape  block_type=mult
  Mult1 : xbsIndex_r4/Mult  precision=Full  arith_type="Signed  (2's comp)"  n_bits=18  bin_pt=17  quantization=Truncate  overflow=Wrap  en=on  latency=mult_latency  use_behavioral_HDL=on  opt=Speed  use_embedded=on  optimum_pipeline=off  pipeline=on  dbl_ovrd=off  use_rpm=off  placement_style=Rectangular shape  block_type=mult
  Register{0..3} (4 alike) : xbsIndex_r4/Register  init=0  rst=off  en=on  dbl_ovrd=off  block_type=register
  coefficient : xbsIndex_r4/Constant  const=factor  gui_display_data_type=Fixed-point  arith_type=Signed (2's comp)  n_bits=coeff_bit_width  bin_pt=coeff_bin_pt  preci_type=Single  exp_width=8  frac_width=24  explicit_period=on  period=1  equ=P=C  opselect=C  inp2=PCIN>>17  opr=+  inp1=P  carry=CIN  dbl_ovrd=off  block_type=constant
  a_out : Outport
  b_out : Outport  Port=2
  c_out : Outport  Port=3
  d_out : Outport  Port=4
  real : Outport  Port=5
  imag : Outport  Port=6
  wires:
  dv_in/1 -> Register0/2, Register1/2, Register2/2, Register3/2, AddSub0/3, AddSub1/3, Mult0/3, Mult1/3
  d/1 -> AddSub1/2, Register3/1
  c/1 -> AddSub0/2, Register2/1
  b/1 -> AddSub1/1, Register1/1
  a/1 -> AddSub0/1, Register0/1
  Register0/1 -> a_out/1
  Register1/1 -> b_out/1
  Register2/1 -> c_out/1
  coefficient/1 -> Mult0/1, Mult1/1
  Register3/1 -> d_out/1
  AddSub0/1 -> Mult0/2
  Mult0/1 -> real/1
  AddSub1/1 -> Mult1/2
  Mult1/1 -> imag/1

== system s_c_nbe_m32k/DDC/dec_fir_async3/fir_col_async4/fir_tap8 ==
  a : Inport
  b : Inport  Port=2
  c : Inport  Port=3
  d : Inport  Port=4
  dv_in : Inport  Port=5
  AddSub0 : xbsIndex_r4/AddSub  mode=Addition  use_carryin=off  use_carryout=off  en=on  latency=add_latency  precision=Full  arith_type="Signed  (2's comp)"  n_bits=18  bin_pt=16  quantization=Truncate  overflow=Wrap  use_behavioral_HDL=on  hw_selection=Fabric  pipelined=off  use_rpm=on  dbl_ovrd=off  block_type=addsub
  AddSub1 : xbsIndex_r4/AddSub  mode=Addition  use_carryin=off  use_carryout=off  en=on  latency=add_latency  precision=Full  arith_type="Signed  (2's comp)"  n_bits=18  bin_pt=16  quantization=Truncate  overflow=Wrap  use_behavioral_HDL=on  hw_selection=Fabric  pipelined=off  use_rpm=on  dbl_ovrd=off  block_type=addsub
  Mult0 : xbsIndex_r4/Mult  precision=Full  arith_type="Signed  (2's comp)"  n_bits=18  bin_pt=17  quantization=Truncate  overflow=Wrap  en=on  latency=mult_latency  use_behavioral_HDL=on  opt=Speed  use_embedded=on  optimum_pipeline=off  pipeline=on  dbl_ovrd=off  use_rpm=off  placement_style=Rectangular shape  block_type=mult
  Mult1 : xbsIndex_r4/Mult  precision=Full  arith_type="Signed  (2's comp)"  n_bits=18  bin_pt=17  quantization=Truncate  overflow=Wrap  en=on  latency=mult_latency  use_behavioral_HDL=on  opt=Speed  use_embedded=on  optimum_pipeline=off  pipeline=on  dbl_ovrd=off  use_rpm=off  placement_style=Rectangular shape  block_type=mult
  Register{0..3} (4 alike) : xbsIndex_r4/Register  init=0  rst=off  en=on  dbl_ovrd=off  block_type=register
  coefficient : xbsIndex_r4/Constant  const=factor  gui_display_data_type=Fixed-point  arith_type=Signed (2's comp)  n_bits=coeff_bit_width  bin_pt=coeff_bin_pt  preci_type=Single  exp_width=8  frac_width=24  explicit_period=on  period=1  equ=P=C  opselect=C  inp2=PCIN>>17  opr=+  inp1=P  carry=CIN  dbl_ovrd=off  block_type=constant
  a_out : Outport
  b_out : Outport  Port=2
  c_out : Outport  Port=3
  d_out : Outport  Port=4
  real : Outport  Port=5
  imag : Outport  Port=6
  wires:
  dv_in/1 -> Register0/2, Register1/2, Register2/2, Register3/2, AddSub0/3, AddSub1/3, Mult0/3, Mult1/3
  d/1 -> AddSub1/2, Register3/1
  c/1 -> AddSub0/2, Register2/1
  b/1 -> AddSub1/1, Register1/1
  a/1 -> AddSub0/1, Register0/1
  Register0/1 -> a_out/1
  Register1/1 -> b_out/1
  Register2/1 -> c_out/1
  coefficient/1 -> Mult0/1, Mult1/1
  Register3/1 -> d_out/1
  AddSub0/1 -> Mult0/2
  Mult0/1 -> real/1
  AddSub1/1 -> Mult1/2
  Mult1/1 -> imag/1
